simulink model "fix_FOC_sync"  (R2025b)
settings: Solver=FixedStepAuto  StartTime=0.0  StopTime=10.0  FixedStep=0.001  RelTol=1e-3
values from neighbouring files (symbols this model uses):
  Dm = 1e-3    (= 0.001)    [motor_param.m]
  Ki_id = wc_c*Rs    (= 380)    [motor_param.m]
  Ki_iq = wc_c*Rs    (= 380)    [motor_param.m]
  Ki_s = 0.041    [motor_param.m]
  Kp_id = wc_c*Ld    (= 10)    [motor_param.m]
  Kp_iq = wc_c*Lq    (= 20)    [motor_param.m]
  Kp_s = 0.0014    [motor_param.m]
  Ld = 0.01    [motor_param.m]
  Lq = 0.02    [motor_param.m]
  p = 2    [motor_param.m]
  Phi = 0.1    [motor_param.m]
libraries: fl_lib x50, nesl_utility x50, slpidlib x15, ee_lib x15, eeTransforms x10
(part 3 of 4)

== system fix_FOC_sync/Subsystem5/Plant/MechSensor ==
  Ideal Rotational Motion Sensor : fl_lib/Mechanical/Mechanical Sensors/Ideal Rotational Motion Sensor  reference=foundation.enum.MeasurementReference.difference  acceleration_port=false  velocity_port=true  position_port=true  wrap_angle=simscape.enum.onoff.off  offset=0 rad
  Ideal Torque Sensor : fl_lib/Mechanical/Mechanical Sensors/Ideal Torque Sensor
  PS-Simulink Converter : nesl_utility/PS-Simulink Converter  PhysicalDomain=network_engine_domain  SubClassName=ps_output  LeftPortType=input  RightPortType=output  PseudoPeriodic=off  Frequencies=[]  VectorFormat=1-D array  Unit=1  AffineConversion=off
  PS-Simulink Converter1 : nesl_utility/PS-Simulink Converter  PhysicalDomain=network_engine_domain  SubClassName=ps_output  LeftPortType=input  RightPortType=output  PseudoPeriodic=off  Frequencies=[]  VectorFormat=1-D array  Unit=1  AffineConversion=off
  PS-Simulink Converter2 : nesl_utility/PS-Simulink Converter  PhysicalDomain=network_engine_domain  SubClassName=ps_output  LeftPortType=input  RightPortType=output  PseudoPeriodic=off  Frequencies=[]  VectorFormat=1-D array  Unit=1  AffineConversion=off
  R1 : PMIOPort  Side=Left
  C1 : PMIOPort  Port=2  Side=Left
  R2 : PMIOPort  Port=3  Side=Right
  C2 : PMIOPort  Port=4  Side=Right
  wm : Outport  VectorParamsAs1DForOutWhenUnconnected=off
  thm : Outport  Port=2  VectorParamsAs1DForOutWhenUnconnected=off
  Tm : Outport  Port=3  VectorParamsAs1DForOutWhenUnconnected=off
  wires:
  PS-Simulink Converter/1 -> thm/1
  PS-Simulink Converter1/1 -> Tm/1
  PS-Simulink Converter2/1 -> wm/1
  connections:
  Ideal Rotational Motion Sensor/RConn3 -- PS-Simulink Converter/LConn1
  Ideal Rotational Motion Sensor/RConn1 -- C2/RConn1 -- C1/RConn1
  Ideal Torque Sensor/LConn1 -- R1/RConn1
  Ideal Torque Sensor/RConn1 -- R2/RConn1 -- Ideal Rotational Motion Sensor/LConn1
  PS-Simulink Converter1/LConn1 -- Ideal Torque Sensor/RConn2
  Ideal Rotational Motion Sensor/RConn2 -- PS-Simulink Converter2/LConn1

== system fix_FOC_sync/Subsystem1/Controller/DriverPeripherals/Break Algebraic Loop ==
  In1 : Inport
  Demux : Demux  Outputs=3
  Mux : Mux  Inputs=3
  Transfer Fcn : TransferFcn  Denominator=[1e-6 1]
  Transfer Fcn1 : TransferFcn  Denominator=[1e-6 1]
  Transfer Fcn2 : TransferFcn  Denominator=[1e-6 1]
  Out1 : Outport
  wires:
  In1/1 -> Demux/1
  Demux/1 -> Transfer Fcn/1
  Transfer Fcn/1 -> Mux/1
  Demux/2 -> Transfer Fcn1/1
  Transfer Fcn1/1 -> Mux/2
  Demux/3 -> Transfer Fcn2/1
  Transfer Fcn2/1 -> Mux/3
  Mux/1 -> Out1/1

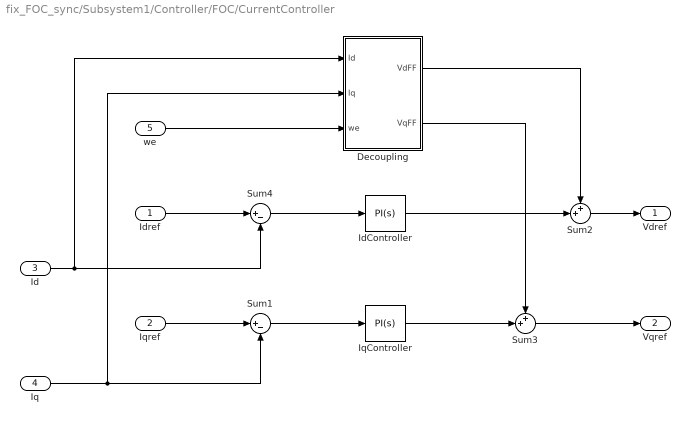
== system fix_FOC_sync/Subsystem1/Controller/FOC/CurrentController ==
  Idref : Inport
  Iqref : Inport  Port=2
  Id : Inport  Port=3
  Iq : Inport  Port=4
  we : Inport  Port=5
  Decoupling : Subsystem
  IdController : slpidlib/PID Controller  Controller=PI  Form=Parallel  TimeDomain=Continuous-time  UseExternalTs=off  SampleTime=-1  IntegratorMethod=Forward Euler  FilterMethod=Forward Euler  ControllerParametersSource=internal  P=Kp_id  I=Ki_id  UseKiTs=off  D=0  UseExternalDerivativeSource=off  N=100  UseFilter=on  TunerSelectOption=Transfer Function Based (PID Tuner App)  InitialConditionSource=internal  InitialConditionForIntegrator=0  InitialConditionForFilter=0  DifferentiatorICPrevScaledInput=0  ExternalReset=none  TrackingMode=off  Kt=1  LimitOutput=off  SatLimitsSource=internal  UpperSaturationLimit=inf  LowerSaturationLimit=-inf  LinearizeAsGain=on  AntiWindupMode=none  Kb=1  LimitIntegrator=off  UpperIntegratorSaturationLimit=inf  LowerIntegratorSaturationLimit=-inf  POutMin=[]  POutMax=[]  IOutMin=[]  IOutMax=[]  DOutMin=[]  DOutMax=[]  NOutMin=[]  NOutMax=[]  SumOutMin=[]  SumOutMax=[]  SaturationOutMin=[]  SaturationOutMax=[]  PParamMin=[]  PParamMax=[]  IParamMin=[]  IParamMax=[]  DParamMin=[]  DParamMax=[]  NParamMin=[]  NParamMax=[]  KbParamMin=[]  KbParamMax=[]  KtParamMin=[]  KtParamMax=[]  KbOutMin=[]  KbOutMax=[]  KtOutMin=[]  KtOutMax=[]  IntegratorOutMin=[]  IntegratorOutMax=[]  FilterOutMin=[]  FilterOutMax=[]  SumI1OutMin=[]  SumI1OutMax=[]  SumI2OutMin=[]  SumI2OutMax=[]  SumI3OutMin=[]  SumI3OutMax=[]  SumI4OutMin=[]  SumI4OutMax=[]  SumDOutMin=[]  SumDOutMax=[]  DifferentiatorOutMin=[]  DifferentiatorOutMax=[]  FilterDiffOutCoefMin=[]  FilterDiffOutCoefMax=[]  ReciprocalOutMin=[]  ReciprocalOutMax=[]  SumDenOutMin=[]  SumDenOutMax=[]  SumNumOutMin=[]  SumNumOutMax=[]  DivideOutMin=[]  DivideOutMax=[]  UdiffTsProdOutMin=[]  UdiffTsProdOutMax=[]  NTsProdOutMin=[]  NTsProdOutMax=[]  UintegralTsProdOutMin=[]  UintegralTsProdOutMax=[]  UngainTsProdOutMin=[]  UngainTsProdOutMax=[]  ClampingZeroOutDataTypeStr=Inherit: Inherit via back propagation  ClampingZeroOutMin=[]  ClampingZeroOutMax=[]  FilterDenConstantOutDataTypeStr=Inherit: Inherit via back propagation  FilterDenConstantOutMin=[]  FilterDenConstantOutMax=[]  PCopyOutDataTypeStr=Inherit: Inherit via back propagation  PCopyOutMin=[]  PCopyOutMax=[]  NCopyOutDataTypeStr=Inherit: Inherit via back propagation  NCopyOutMin=[]  NCopyOutMax=[]  IntegratorContinuousStateAttributes=''  IntegratorStateMustResolveToSignalObject=off  IntegratorRTWStateStorageClass=Auto  FilterContinuousStateAttributes=''  FilterStateMustResolveToSignalObject=off  FilterRTWStateStorageClass=Auto  ParallelPVariant=InternalParameters  IdealPVariant=Disabled  IVariant=InternalParameters  DVariant=Disabled  IntegratorVariant=Continuous  SatVariant=Disabled  AWVariant=Passthrough  PCopyVariant=Disabled  TRVariant=Disabled  FdbkBlocksVariant=Forward  IdealPFdbkVariant=Disabled  SatFdbkVariant=Disabled  DerivativeFilterVariant=Disabled  NVariant=Disabled  NCopyVariant=Disabled_SignalSpec  FilterICVariant=Disabled  IntegratorICVariant=InternalICs  ExternalResetVariant=Disabled  TRSumVariant=Passthrough  SumFdbkVariant=Disabled  SumVariant=Sum_PI  TsampFilterVariant=InternalTs  TsampNgainVariant=Passthrough  TsampIntegralVariant=Disabled_SignalSpec  ExternalSaturationOutDataTypeStr=Inherit: Same as second input  DerivativeSourceVariant=Disabled  PreIntVariant=InternalPreInt
  IqController : slpidlib/PID Controller  Controller=PI  Form=Parallel  TimeDomain=Continuous-time  UseExternalTs=off  SampleTime=-1  IntegratorMethod=Forward Euler  FilterMethod=Forward Euler  ControllerParametersSource=internal  P=Kp_iq  I=Ki_iq  UseKiTs=off  D=0  UseExternalDerivativeSource=off  N=100  UseFilter=on  TunerSelectOption=Transfer Function Based (PID Tuner App)  InitialConditionSource=internal  InitialConditionForIntegrator=0  InitialConditionForFilter=0  DifferentiatorICPrevScaledInput=0  ExternalReset=none  TrackingMode=off  Kt=1  LimitOutput=off  SatLimitsSource=internal  UpperSaturationLimit=inf  LowerSaturationLimit=-inf  LinearizeAsGain=on  AntiWindupMode=none  Kb=1  LimitIntegrator=off  UpperIntegratorSaturationLimit=inf  LowerIntegratorSaturationLimit=-inf  POutMin=[]  POutMax=[]  IOutMin=[]  IOutMax=[]  DOutMin=[]  DOutMax=[]  NOutMin=[]  NOutMax=[]  SumOutMin=[]  SumOutMax=[]  SaturationOutMin=[]  SaturationOutMax=[]  PParamMin=[]  PParamMax=[]  IParamMin=[]  IParamMax=[]  DParamMin=[]  DParamMax=[]  NParamMin=[]  NParamMax=[]  KbParamMin=[]  KbParamMax=[]  KtParamMin=[]  KtParamMax=[]  KbOutMin=[]  KbOutMax=[]  KtOutMin=[]  KtOutMax=[]  IntegratorOutMin=[]  IntegratorOutMax=[]  FilterOutMin=[]  FilterOutMax=[]  SumI1OutMin=[]  SumI1OutMax=[]  SumI2OutMin=[]  SumI2OutMax=[]  SumI3OutMin=[]  SumI3OutMax=[]  SumI4OutMin=[]  SumI4OutMax=[]  SumDOutMin=[]  SumDOutMax=[]  DifferentiatorOutMin=[]  DifferentiatorOutMax=[]  FilterDiffOutCoefMin=[]  FilterDiffOutCoefMax=[]  ReciprocalOutMin=[]  ReciprocalOutMax=[]  SumDenOutMin=[]  SumDenOutMax=[]  SumNumOutMin=[]  SumNumOutMax=[]  DivideOutMin=[]  DivideOutMax=[]  UdiffTsProdOutMin=[]  UdiffTsProdOutMax=[]  NTsProdOutMin=[]  NTsProdOutMax=[]  UintegralTsProdOutMin=[]  UintegralTsProdOutMax=[]  UngainTsProdOutMin=[]  UngainTsProdOutMax=[]  ClampingZeroOutDataTypeStr=Inherit: Inherit via back propagation  ClampingZeroOutMin=[]  ClampingZeroOutMax=[]  FilterDenConstantOutDataTypeStr=Inherit: Inherit via back propagation  FilterDenConstantOutMin=[]  FilterDenConstantOutMax=[]  PCopyOutDataTypeStr=Inherit: Inherit via back propagation  PCopyOutMin=[]  PCopyOutMax=[]  NCopyOutDataTypeStr=Inherit: Inherit via back propagation  NCopyOutMin=[]  NCopyOutMax=[]  IntegratorContinuousStateAttributes=''  IntegratorStateMustResolveToSignalObject=off  IntegratorRTWStateStorageClass=Auto  FilterContinuousStateAttributes=''  FilterStateMustResolveToSignalObject=off  FilterRTWStateStorageClass=Auto  ParallelPVariant=InternalParameters  IdealPVariant=Disabled  IVariant=InternalParameters  DVariant=Disabled  IntegratorVariant=Continuous  SatVariant=Disabled  AWVariant=Passthrough  PCopyVariant=Disabled  TRVariant=Disabled  FdbkBlocksVariant=Forward  IdealPFdbkVariant=Disabled  SatFdbkVariant=Disabled  DerivativeFilterVariant=Disabled  NVariant=Disabled  NCopyVariant=Disabled_SignalSpec  FilterICVariant=Disabled  IntegratorICVariant=InternalICs  ExternalResetVariant=Disabled  TRSumVariant=Passthrough  SumFdbkVariant=Disabled  SumVariant=Sum_PI  TsampFilterVariant=InternalTs  TsampNgainVariant=Passthrough  TsampIntegralVariant=Disabled_SignalSpec  ExternalSaturationOutDataTypeStr=Inherit: Same as second input  DerivativeSourceVariant=Disabled  PreIntVariant=InternalPreInt
  Sum1 : Sum  Inputs=|+-
  Sum2 : Sum  Inputs=++|
  Sum3 : Sum  Inputs=++|
  Sum4 : Sum  Inputs=|+-
  Vdref : Outport  VectorParamsAs1DForOutWhenUnconnected=off
  Vqref : Outport  Port=2  VectorParamsAs1DForOutWhenUnconnected=off
  wires:
  we/1 -> Decoupling/3(we)
  Idref/1 -> Sum4/1
  Sum2/1 -> Vdref/1
  Sum3/1 -> Vqref/1
  Iqref/1 -> Sum1/1
  Iq/1 -> Decoupling/2(Iq), Sum1/2
  Id/1 -> Decoupling/1(Id), Sum4/2
  Sum4/1 -> IdController/1
  Sum1/1 -> IqController/1
  Decoupling/2(VqFF) -> Sum3/1
  Decoupling/1(VdFF) -> Sum2/1
  IdController/1 -> Sum2/2
  IqController/1 -> Sum3/2

== system fix_FOC_sync/Subsystem1/Controller/FOC/VelocityController ==
  wmref : Inport
  wm : Inport  Port=2
  Gain : Gain  Gain=1/(3/2*p*Phi)
  PIDController : slpidlib/PID Controller  Controller=PI  Form=Parallel  TimeDomain=Continuous-time  UseExternalTs=off  SampleTime=-1  IntegratorMethod=Forward Euler  FilterMethod=Forward Euler  ControllerParametersSource=internal  P=Kp_s  I=Ki_s  UseKiTs=off  D=0  UseExternalDerivativeSource=off  N=100  UseFilter=on  TunerSelectOption=Transfer Function Based (PID Tuner App)  InitialConditionSource=internal  InitialConditionForIntegrator=0  InitialConditionForFilter=0  DifferentiatorICPrevScaledInput=0  ExternalReset=none  TrackingMode=off  Kt=1  LimitOutput=off  SatLimitsSource=internal  UpperSaturationLimit=inf  LowerSaturationLimit=-inf  LinearizeAsGain=on  AntiWindupMode=none  Kb=1  LimitIntegrator=off  UpperIntegratorSaturationLimit=inf  LowerIntegratorSaturationLimit=-inf  POutMin=[]  POutMax=[]  IOutMin=[]  IOutMax=[]  DOutMin=[]  DOutMax=[]  NOutMin=[]  NOutMax=[]  SumOutMin=[]  SumOutMax=[]  SaturationOutMin=[]  SaturationOutMax=[]  PParamMin=[]  PParamMax=[]  IParamMin=[]  IParamMax=[]  DParamMin=[]  DParamMax=[]  NParamMin=[]  NParamMax=[]  KbParamMin=[]  KbParamMax=[]  KtParamMin=[]  KtParamMax=[]  KbOutMin=[]  KbOutMax=[]  KtOutMin=[]  KtOutMax=[]  IntegratorOutMin=[]  IntegratorOutMax=[]  FilterOutMin=[]  FilterOutMax=[]  SumI1OutMin=[]  SumI1OutMax=[]  SumI2OutMin=[]  SumI2OutMax=[]  SumI3OutMin=[]  SumI3OutMax=[]  SumI4OutMin=[]  SumI4OutMax=[]  SumDOutMin=[]  SumDOutMax=[]  DifferentiatorOutMin=[]  DifferentiatorOutMax=[]  FilterDiffOutCoefMin=[]  FilterDiffOutCoefMax=[]  ReciprocalOutMin=[]  ReciprocalOutMax=[]  SumDenOutMin=[]  SumDenOutMax=[]  SumNumOutMin=[]  SumNumOutMax=[]  DivideOutMin=[]  DivideOutMax=[]  UdiffTsProdOutMin=[]  UdiffTsProdOutMax=[]  NTsProdOutMin=[]  NTsProdOutMax=[]  UintegralTsProdOutMin=[]  UintegralTsProdOutMax=[]  UngainTsProdOutMin=[]  UngainTsProdOutMax=[]  ClampingZeroOutDataTypeStr=Inherit: Inherit via back propagation  ClampingZeroOutMin=[]  ClampingZeroOutMax=[]  FilterDenConstantOutDataTypeStr=Inherit: Inherit via back propagation  FilterDenConstantOutMin=[]  FilterDenConstantOutMax=[]  PCopyOutDataTypeStr=Inherit: Inherit via back propagation  PCopyOutMin=[]  PCopyOutMax=[]  NCopyOutDataTypeStr=Inherit: Inherit via back propagation  NCopyOutMin=[]  NCopyOutMax=[]  IntegratorContinuousStateAttributes=''  IntegratorStateMustResolveToSignalObject=off  IntegratorRTWStateStorageClass=Auto  FilterContinuousStateAttributes=''  FilterStateMustResolveToSignalObject=off  FilterRTWStateStorageClass=Auto  ParallelPVariant=InternalParameters  IdealPVariant=Disabled  IVariant=InternalParameters  DVariant=Disabled  IntegratorVariant=Continuous  SatVariant=Disabled  AWVariant=Passthrough  PCopyVariant=Disabled  TRVariant=Disabled  FdbkBlocksVariant=Forward  IdealPFdbkVariant=Disabled  SatFdbkVariant=Disabled  DerivativeFilterVariant=Disabled  NVariant=Disabled  NCopyVariant=Disabled_SignalSpec  FilterICVariant=Disabled  IntegratorICVariant=InternalICs  ExternalResetVariant=Disabled  TRSumVariant=Passthrough  SumFdbkVariant=Disabled  SumVariant=Sum_PI  TsampFilterVariant=InternalTs  TsampNgainVariant=Passthrough  TsampIntegralVariant=Disabled_SignalSpec  ExternalSaturationOutDataTypeStr=Inherit: Same as second input  DerivativeSourceVariant=Disabled  PreIntVariant=InternalPreInt
  Sum : Sum  Inputs=|+-
  Iqref : Outport  VectorParamsAs1DForOutWhenUnconnected=off
  wires:
  Gain/1 -> Iqref/1
  wmref/1 -> Sum/1
  wm/1 -> Sum/2
  Sum/1 -> PIDController/1
  PIDController/1 -> Gain/1

== system fix_FOC_sync/Subsystem1/Controller/FOC/abc2dq ==
  Iabc : Inport
  thetae : Inport  Port=2
  Demux1 : Demux  Outputs=3
  Park Transform : eeTransforms/Park Transform  AxisAlignment=D-axis  PowerInvariant=off
  Terminator : Terminator
  Id : Outport  VectorParamsAs1DForOutWhenUnconnected=off
  Iq : Outport  Port=2  VectorParamsAs1DForOutWhenUnconnected=off
  wires:
  Iabc/1 -> Park Transform/1
  thetae/1 -> Park Transform/2
  Demux1/3 -> Terminator/1
  Park Transform/1 -> Demux1/1
  Demux1/1 -> Id/1
  Demux1/2 -> Iq/1

== system fix_FOC_sync/Subsystem1/Controller/FOC/dq2abc ==
  Vd : Inport
  Vq : Inport  Port=2
  thetae : Inport  Port=3
  Constant : Constant  Value=0
  Inverse Park Transform : eeTransforms/Inverse Park Transform  AxisAlignment=D-axis  PowerInvariant=off
  Mux : Mux  Inputs=3
  Vabc : Outport  VectorParamsAs1DForOutWhenUnconnected=off
  wires:
  thetae/1 -> Inverse Park Transform/2
  Constant/1 -> Mux/3
  Mux/1 -> Inverse Park Transform/1
  Vd/1 -> Mux/1
  Inverse Park Transform/1 -> Vabc/1
  Vq/1 -> Mux/2

== system fix_FOC_sync/Subsystem1/Controller/FOC/thm2the ==
  thm : Inport
  Constant : Constant  Value=2*pi
  Mod : Math  Operator=mod  SignedPower=on
  PolePairs : Gain  Gain=p
  the : Outport  VectorParamsAs1DForOutWhenUnconnected=off
  wires:
  Constant/1 -> Mod/2
  PolePairs/1 -> Mod/1
  Mod/1 -> the/1
  thm/1 -> PolePairs/1

== system fix_FOC_sync/Subsystem1/Controller/FOC/wm2we ==
  wm : Inport
  PolePairs : Gain  Gain=p
  we : Outport  VectorParamsAs1DForOutWhenUnconnected=off
  wires:
  wm/1 -> PolePairs/1
  PolePairs/1 -> we/1

== system fix_FOC_sync/Subsystem2/Controller/DriverPeripherals/Break Algebraic Loop ==
  In1 : Inport
  Demux : Demux  Outputs=3
  Mux : Mux  Inputs=3
  Transfer Fcn : TransferFcn  Denominator=[1e-6 1]
  Transfer Fcn1 : TransferFcn  Denominator=[1e-6 1]
  Transfer Fcn2 : TransferFcn  Denominator=[1e-6 1]
  Out1 : Outport
  wires:
  In1/1 -> Demux/1
  Demux/1 -> Transfer Fcn/1
  Transfer Fcn/1 -> Mux/1
  Demux/2 -> Transfer Fcn1/1
  Transfer Fcn1/1 -> Mux/2
  Demux/3 -> Transfer Fcn2/1
  Transfer Fcn2/1 -> Mux/3
  Mux/1 -> Out1/1

== system fix_FOC_sync/Subsystem2/Controller/FOC/CurrentController ==
  Idref : Inport
  Iqref : Inport  Port=2
  Id : Inport  Port=3
  Iq : Inport  Port=4
  we : Inport  Port=5
  Decoupling : Subsystem
  IdController : slpidlib/PID Controller  Controller=PI  Form=Parallel  TimeDomain=Continuous-time  UseExternalTs=off  SampleTime=-1  IntegratorMethod=Forward Euler  FilterMethod=Forward Euler  ControllerParametersSource=internal  P=Kp_id  I=Ki_id  UseKiTs=off  D=0  UseExternalDerivativeSource=off  N=100  UseFilter=on  TunerSelectOption=Transfer Function Based (PID Tuner App)  InitialConditionSource=internal  InitialConditionForIntegrator=0  InitialConditionForFilter=0  DifferentiatorICPrevScaledInput=0  ExternalReset=none  TrackingMode=off  Kt=1  LimitOutput=off  SatLimitsSource=internal  UpperSaturationLimit=inf  LowerSaturationLimit=-inf  LinearizeAsGain=on  AntiWindupMode=none  Kb=1  LimitIntegrator=off  UpperIntegratorSaturationLimit=inf  LowerIntegratorSaturationLimit=-inf  POutMin=[]  POutMax=[]  IOutMin=[]  IOutMax=[]  DOutMin=[]  DOutMax=[]  NOutMin=[]  NOutMax=[]  SumOutMin=[]  SumOutMax=[]  SaturationOutMin=[]  SaturationOutMax=[]  PParamMin=[]  PParamMax=[]  IParamMin=[]  IParamMax=[]  DParamMin=[]  DParamMax=[]  NParamMin=[]  NParamMax=[]  KbParamMin=[]  KbParamMax=[]  KtParamMin=[]  KtParamMax=[]  KbOutMin=[]  KbOutMax=[]  KtOutMin=[]  KtOutMax=[]  IntegratorOutMin=[]  IntegratorOutMax=[]  FilterOutMin=[]  FilterOutMax=[]  SumI1OutMin=[]  SumI1OutMax=[]  SumI2OutMin=[]  SumI2OutMax=[]  SumI3OutMin=[]  SumI3OutMax=[]  SumI4OutMin=[]  SumI4OutMax=[]  SumDOutMin=[]  SumDOutMax=[]  DifferentiatorOutMin=[]  DifferentiatorOutMax=[]  FilterDiffOutCoefMin=[]  FilterDiffOutCoefMax=[]  ReciprocalOutMin=[]  ReciprocalOutMax=[]  SumDenOutMin=[]  SumDenOutMax=[]  SumNumOutMin=[]  SumNumOutMax=[]  DivideOutMin=[]  DivideOutMax=[]  UdiffTsProdOutMin=[]  UdiffTsProdOutMax=[]  NTsProdOutMin=[]  NTsProdOutMax=[]  UintegralTsProdOutMin=[]  UintegralTsProdOutMax=[]  UngainTsProdOutMin=[]  UngainTsProdOutMax=[]  ClampingZeroOutDataTypeStr=Inherit: Inherit via back propagation  ClampingZeroOutMin=[]  ClampingZeroOutMax=[]  FilterDenConstantOutDataTypeStr=Inherit: Inherit via back propagation  FilterDenConstantOutMin=[]  FilterDenConstantOutMax=[]  PCopyOutDataTypeStr=Inherit: Inherit via back propagation  PCopyOutMin=[]  PCopyOutMax=[]  NCopyOutDataTypeStr=Inherit: Inherit via back propagation  NCopyOutMin=[]  NCopyOutMax=[]  IntegratorContinuousStateAttributes=''  IntegratorStateMustResolveToSignalObject=off  IntegratorRTWStateStorageClass=Auto  FilterContinuousStateAttributes=''  FilterStateMustResolveToSignalObject=off  FilterRTWStateStorageClass=Auto  ParallelPVariant=InternalParameters  IdealPVariant=Disabled  IVariant=InternalParameters  DVariant=Disabled  IntegratorVariant=Continuous  SatVariant=Disabled  AWVariant=Passthrough  PCopyVariant=Disabled  TRVariant=Disabled  FdbkBlocksVariant=Forward  IdealPFdbkVariant=Disabled  SatFdbkVariant=Disabled  DerivativeFilterVariant=Disabled  NVariant=Disabled  NCopyVariant=Disabled_SignalSpec  FilterICVariant=Disabled  IntegratorICVariant=InternalICs  ExternalResetVariant=Disabled  TRSumVariant=Passthrough  SumFdbkVariant=Disabled  SumVariant=Sum_PI  TsampFilterVariant=InternalTs  TsampNgainVariant=Passthrough  TsampIntegralVariant=Disabled_SignalSpec  ExternalSaturationOutDataTypeStr=Inherit: Same as second input  DerivativeSourceVariant=Disabled  PreIntVariant=InternalPreInt
  IqController : slpidlib/PID Controller  Controller=PI  Form=Parallel  TimeDomain=Continuous-time  UseExternalTs=off  SampleTime=-1  IntegratorMethod=Forward Euler  FilterMethod=Forward Euler  ControllerParametersSource=internal  P=Kp_iq  I=Ki_iq  UseKiTs=off  D=0  UseExternalDerivativeSource=off  N=100  UseFilter=on  TunerSelectOption=Transfer Function Based (PID Tuner App)  InitialConditionSource=internal  InitialConditionForIntegrator=0  InitialConditionForFilter=0  DifferentiatorICPrevScaledInput=0  ExternalReset=none  TrackingMode=off  Kt=1  LimitOutput=off  SatLimitsSource=internal  UpperSaturationLimit=inf  LowerSaturationLimit=-inf  LinearizeAsGain=on  AntiWindupMode=none  Kb=1  LimitIntegrator=off  UpperIntegratorSaturationLimit=inf  LowerIntegratorSaturationLimit=-inf  POutMin=[]  POutMax=[]  IOutMin=[]  IOutMax=[]  DOutMin=[]  DOutMax=[]  NOutMin=[]  NOutMax=[]  SumOutMin=[]  SumOutMax=[]  SaturationOutMin=[]  SaturationOutMax=[]  PParamMin=[]  PParamMax=[]  IParamMin=[]  IParamMax=[]  DParamMin=[]  DParamMax=[]  NParamMin=[]  NParamMax=[]  KbParamMin=[]  KbParamMax=[]  KtParamMin=[]  KtParamMax=[]  KbOutMin=[]  KbOutMax=[]  KtOutMin=[]  KtOutMax=[]  IntegratorOutMin=[]  IntegratorOutMax=[]  FilterOutMin=[]  FilterOutMax=[]  SumI1OutMin=[]  SumI1OutMax=[]  SumI2OutMin=[]  SumI2OutMax=[]  SumI3OutMin=[]  SumI3OutMax=[]  SumI4OutMin=[]  SumI4OutMax=[]  SumDOutMin=[]  SumDOutMax=[]  DifferentiatorOutMin=[]  DifferentiatorOutMax=[]  FilterDiffOutCoefMin=[]  FilterDiffOutCoefMax=[]  ReciprocalOutMin=[]  ReciprocalOutMax=[]  SumDenOutMin=[]  SumDenOutMax=[]  SumNumOutMin=[]  SumNumOutMax=[]  DivideOutMin=[]  DivideOutMax=[]  UdiffTsProdOutMin=[]  UdiffTsProdOutMax=[]  NTsProdOutMin=[]  NTsProdOutMax=[]  UintegralTsProdOutMin=[]  UintegralTsProdOutMax=[]  UngainTsProdOutMin=[]  UngainTsProdOutMax=[]  ClampingZeroOutDataTypeStr=Inherit: Inherit via back propagation  ClampingZeroOutMin=[]  ClampingZeroOutMax=[]  FilterDenConstantOutDataTypeStr=Inherit: Inherit via back propagation  FilterDenConstantOutMin=[]  FilterDenConstantOutMax=[]  PCopyOutDataTypeStr=Inherit: Inherit via back propagation  PCopyOutMin=[]  PCopyOutMax=[]  NCopyOutDataTypeStr=Inherit: Inherit via back propagation  NCopyOutMin=[]  NCopyOutMax=[]  IntegratorContinuousStateAttributes=''  IntegratorStateMustResolveToSignalObject=off  IntegratorRTWStateStorageClass=Auto  FilterContinuousStateAttributes=''  FilterStateMustResolveToSignalObject=off  FilterRTWStateStorageClass=Auto  ParallelPVariant=InternalParameters  IdealPVariant=Disabled  IVariant=InternalParameters  DVariant=Disabled  IntegratorVariant=Continuous  SatVariant=Disabled  AWVariant=Passthrough  PCopyVariant=Disabled  TRVariant=Disabled  FdbkBlocksVariant=Forward  IdealPFdbkVariant=Disabled  SatFdbkVariant=Disabled  DerivativeFilterVariant=Disabled  NVariant=Disabled  NCopyVariant=Disabled_SignalSpec  FilterICVariant=Disabled  IntegratorICVariant=InternalICs  ExternalResetVariant=Disabled  TRSumVariant=Passthrough  SumFdbkVariant=Disabled  SumVariant=Sum_PI  TsampFilterVariant=InternalTs  TsampNgainVariant=Passthrough  TsampIntegralVariant=Disabled_SignalSpec  ExternalSaturationOutDataTypeStr=Inherit: Same as second input  DerivativeSourceVariant=Disabled  PreIntVariant=InternalPreInt
  Sum1 : Sum  Inputs=|+-
  Sum2 : Sum  Inputs=++|
  Sum3 : Sum  Inputs=++|
  Sum4 : Sum  Inputs=|+-
  Vdref : Outport  VectorParamsAs1DForOutWhenUnconnected=off
  Vqref : Outport  Port=2  VectorParamsAs1DForOutWhenUnconnected=off
  wires:
  we/1 -> Decoupling/3(we)
  Idref/1 -> Sum4/1
  Sum2/1 -> Vdref/1
  Sum3/1 -> Vqref/1
  Iqref/1 -> Sum1/1
  Iq/1 -> Decoupling/2(Iq), Sum1/2
  Id/1 -> Decoupling/1(Id), Sum4/2
  Sum4/1 -> IdController/1
  Sum1/1 -> IqController/1
  Decoupling/2(VqFF) -> Sum3/1
  Decoupling/1(VdFF) -> Sum2/1
  IdController/1 -> Sum2/2
  IqController/1 -> Sum3/2

== system fix_FOC_sync/Subsystem2/Controller/FOC/VelocityController ==
  wmref : Inport
  wm : Inport  Port=2
  Gain : Gain  Gain=1/(3/2*p*Phi)
  PIDController : slpidlib/PID Controller  Controller=PI  Form=Parallel  TimeDomain=Continuous-time  UseExternalTs=off  SampleTime=-1  IntegratorMethod=Forward Euler  FilterMethod=Forward Euler  ControllerParametersSource=internal  P=Kp_s  I=Ki_s  UseKiTs=off  D=0  UseExternalDerivativeSource=off  N=100  UseFilter=on  TunerSelectOption=Transfer Function Based (PID Tuner App)  InitialConditionSource=internal  InitialConditionForIntegrator=0  InitialConditionForFilter=0  DifferentiatorICPrevScaledInput=0  ExternalReset=none  TrackingMode=off  Kt=1  LimitOutput=off  SatLimitsSource=internal  UpperSaturationLimit=inf  LowerSaturationLimit=-inf  LinearizeAsGain=on  AntiWindupMode=none  Kb=1  LimitIntegrator=off  UpperIntegratorSaturationLimit=inf  LowerIntegratorSaturationLimit=-inf  POutMin=[]  POutMax=[]  IOutMin=[]  IOutMax=[]  DOutMin=[]  DOutMax=[]  NOutMin=[]  NOutMax=[]  SumOutMin=[]  SumOutMax=[]  SaturationOutMin=[]  SaturationOutMax=[]  PParamMin=[]  PParamMax=[]  IParamMin=[]  IParamMax=[]  DParamMin=[]  DParamMax=[]  NParamMin=[]  NParamMax=[]  KbParamMin=[]  KbParamMax=[]  KtParamMin=[]  KtParamMax=[]  KbOutMin=[]  KbOutMax=[]  KtOutMin=[]  KtOutMax=[]  IntegratorOutMin=[]  IntegratorOutMax=[]  FilterOutMin=[]  FilterOutMax=[]  SumI1OutMin=[]  SumI1OutMax=[]  SumI2OutMin=[]  SumI2OutMax=[]  SumI3OutMin=[]  SumI3OutMax=[]  SumI4OutMin=[]  SumI4OutMax=[]  SumDOutMin=[]  SumDOutMax=[]  DifferentiatorOutMin=[]  DifferentiatorOutMax=[]  FilterDiffOutCoefMin=[]  FilterDiffOutCoefMax=[]  ReciprocalOutMin=[]  ReciprocalOutMax=[]  SumDenOutMin=[]  SumDenOutMax=[]  SumNumOutMin=[]  SumNumOutMax=[]  DivideOutMin=[]  DivideOutMax=[]  UdiffTsProdOutMin=[]  UdiffTsProdOutMax=[]  NTsProdOutMin=[]  NTsProdOutMax=[]  UintegralTsProdOutMin=[]  UintegralTsProdOutMax=[]  UngainTsProdOutMin=[]  UngainTsProdOutMax=[]  ClampingZeroOutDataTypeStr=Inherit: Inherit via back propagation  ClampingZeroOutMin=[]  ClampingZeroOutMax=[]  FilterDenConstantOutDataTypeStr=Inherit: Inherit via back propagation  FilterDenConstantOutMin=[]  FilterDenConstantOutMax=[]  PCopyOutDataTypeStr=Inherit: Inherit via back propagation  PCopyOutMin=[]  PCopyOutMax=[]  NCopyOutDataTypeStr=Inherit: Inherit via back propagation  NCopyOutMin=[]  NCopyOutMax=[]  IntegratorContinuousStateAttributes=''  IntegratorStateMustResolveToSignalObject=off  IntegratorRTWStateStorageClass=Auto  FilterContinuousStateAttributes=''  FilterStateMustResolveToSignalObject=off  FilterRTWStateStorageClass=Auto  ParallelPVariant=InternalParameters  IdealPVariant=Disabled  IVariant=InternalParameters  DVariant=Disabled  IntegratorVariant=Continuous  SatVariant=Disabled  AWVariant=Passthrough  PCopyVariant=Disabled  TRVariant=Disabled  FdbkBlocksVariant=Forward  IdealPFdbkVariant=Disabled  SatFdbkVariant=Disabled  DerivativeFilterVariant=Disabled  NVariant=Disabled  NCopyVariant=Disabled_SignalSpec  FilterICVariant=Disabled  IntegratorICVariant=InternalICs  ExternalResetVariant=Disabled  TRSumVariant=Passthrough  SumFdbkVariant=Disabled  SumVariant=Sum_PI  TsampFilterVariant=InternalTs  TsampNgainVariant=Passthrough  TsampIntegralVariant=Disabled_SignalSpec  ExternalSaturationOutDataTypeStr=Inherit: Same as second input  DerivativeSourceVariant=Disabled  PreIntVariant=InternalPreInt
  Sum : Sum  Inputs=|+-
  Iqref : Outport  VectorParamsAs1DForOutWhenUnconnected=off
  wires:
  PIDController/1 -> Gain/1
  Gain/1 -> Iqref/1
  wmref/1 -> Sum/1
  Sum/1 -> PIDController/1
  wm/1 -> Sum/2

== system fix_FOC_sync/Subsystem2/Controller/FOC/abc2dq ==
  Iabc : Inport
  thetae : Inport  Port=2
  Demux1 : Demux  Outputs=3
  Park Transform : eeTransforms/Park Transform  AxisAlignment=D-axis  PowerInvariant=off
  Terminator : Terminator
  Id : Outport  VectorParamsAs1DForOutWhenUnconnected=off
  Iq : Outport  Port=2  VectorParamsAs1DForOutWhenUnconnected=off
  wires:
  Iabc/1 -> Park Transform/1
  thetae/1 -> Park Transform/2
  Demux1/3 -> Terminator/1
  Park Transform/1 -> Demux1/1
  Demux1/1 -> Id/1
  Demux1/2 -> Iq/1

== system fix_FOC_sync/Subsystem2/Controller/FOC/dq2abc ==
  Vd : Inport
  Vq : Inport  Port=2
  thetae : Inport  Port=3
  Constant : Constant  Value=0
  Inverse Park Transform : eeTransforms/Inverse Park Transform  AxisAlignment=D-axis  PowerInvariant=off
  Mux : Mux  Inputs=3
  Vabc : Outport  VectorParamsAs1DForOutWhenUnconnected=off
  wires:
  thetae/1 -> Inverse Park Transform/2
  Constant/1 -> Mux/3
  Mux/1 -> Inverse Park Transform/1
  Vd/1 -> Mux/1
  Inverse Park Transform/1 -> Vabc/1
  Vq/1 -> Mux/2

== system fix_FOC_sync/Subsystem2/Controller/FOC/thm2the ==
  thm : Inport
  Constant : Constant  Value=2*pi
  Mod : Math  Operator=mod  SignedPower=on
  PolePairs : Gain  Gain=p
  the : Outport  VectorParamsAs1DForOutWhenUnconnected=off
  wires:
  Constant/1 -> Mod/2
  PolePairs/1 -> Mod/1
  Mod/1 -> the/1
  thm/1 -> PolePairs/1

== system fix_FOC_sync/Subsystem2/Controller/FOC/wm2we ==
  wm : Inport
  PolePairs : Gain  Gain=p
  we : Outport  VectorParamsAs1DForOutWhenUnconnected=off
  wires:
  wm/1 -> PolePairs/1
  PolePairs/1 -> we/1

== system fix_FOC_sync/Subsystem3/Controller/DriverPeripherals/Break Algebraic Loop ==
  In1 : Inport
  Demux : Demux  Outputs=3
  Mux : Mux  Inputs=3
  Transfer Fcn : TransferFcn  Denominator=[1e-6 1]
  Transfer Fcn1 : TransferFcn  Denominator=[1e-6 1]
  Transfer Fcn2 : TransferFcn  Denominator=[1e-6 1]
  Out1 : Outport
  wires:
  In1/1 -> Demux/1
  Demux/1 -> Transfer Fcn/1
  Transfer Fcn/1 -> Mux/1
  Demux/2 -> Transfer Fcn1/1
  Transfer Fcn1/1 -> Mux/2
  Demux/3 -> Transfer Fcn2/1
  Transfer Fcn2/1 -> Mux/3
  Mux/1 -> Out1/1

== system fix_FOC_sync/Subsystem3/Controller/FOC/CurrentController ==
  Idref : Inport
  Iqref : Inport  Port=2
  Id : Inport  Port=3
  Iq : Inport  Port=4
  we : Inport  Port=5
  Decoupling : Subsystem
  IdController : slpidlib/PID Controller  Controller=PI  Form=Parallel  TimeDomain=Continuous-time  UseExternalTs=off  SampleTime=-1  IntegratorMethod=Forward Euler  FilterMethod=Forward Euler  ControllerParametersSource=internal  P=Kp_id  I=Ki_id  UseKiTs=off  D=0  UseExternalDerivativeSource=off  N=100  UseFilter=on  TunerSelectOption=Transfer Function Based (PID Tuner App)  InitialConditionSource=internal  InitialConditionForIntegrator=0  InitialConditionForFilter=0  DifferentiatorICPrevScaledInput=0  ExternalReset=none  TrackingMode=off  Kt=1  LimitOutput=off  SatLimitsSource=internal  UpperSaturationLimit=inf  LowerSaturationLimit=-inf  LinearizeAsGain=on  AntiWindupMode=none  Kb=1  LimitIntegrator=off  UpperIntegratorSaturationLimit=inf  LowerIntegratorSaturationLimit=-inf  POutMin=[]  POutMax=[]  IOutMin=[]  IOutMax=[]  DOutMin=[]  DOutMax=[]  NOutMin=[]  NOutMax=[]  SumOutMin=[]  SumOutMax=[]  SaturationOutMin=[]  SaturationOutMax=[]  PParamMin=[]  PParamMax=[]  IParamMin=[]  IParamMax=[]  DParamMin=[]  DParamMax=[]  NParamMin=[]  NParamMax=[]  KbParamMin=[]  KbParamMax=[]  KtParamMin=[]  KtParamMax=[]  KbOutMin=[]  KbOutMax=[]  KtOutMin=[]  KtOutMax=[]  IntegratorOutMin=[]  IntegratorOutMax=[]  FilterOutMin=[]  FilterOutMax=[]  SumI1OutMin=[]  SumI1OutMax=[]  SumI2OutMin=[]  SumI2OutMax=[]  SumI3OutMin=[]  SumI3OutMax=[]  SumI4OutMin=[]  SumI4OutMax=[]  SumDOutMin=[]  SumDOutMax=[]  DifferentiatorOutMin=[]  DifferentiatorOutMax=[]  FilterDiffOutCoefMin=[]  FilterDiffOutCoefMax=[]  ReciprocalOutMin=[]  ReciprocalOutMax=[]  SumDenOutMin=[]  SumDenOutMax=[]  SumNumOutMin=[]  SumNumOutMax=[]  DivideOutMin=[]  DivideOutMax=[]  UdiffTsProdOutMin=[]  UdiffTsProdOutMax=[]  NTsProdOutMin=[]  NTsProdOutMax=[]  UintegralTsProdOutMin=[]  UintegralTsProdOutMax=[]  UngainTsProdOutMin=[]  UngainTsProdOutMax=[]  ClampingZeroOutDataTypeStr=Inherit: Inherit via back propagation  ClampingZeroOutMin=[]  ClampingZeroOutMax=[]  FilterDenConstantOutDataTypeStr=Inherit: Inherit via back propagation  FilterDenConstantOutMin=[]  FilterDenConstantOutMax=[]  PCopyOutDataTypeStr=Inherit: Inherit via back propagation  PCopyOutMin=[]  PCopyOutMax=[]  NCopyOutDataTypeStr=Inherit: Inherit via back propagation  NCopyOutMin=[]  NCopyOutMax=[]  IntegratorContinuousStateAttributes=''  IntegratorStateMustResolveToSignalObject=off  IntegratorRTWStateStorageClass=Auto  FilterContinuousStateAttributes=''  FilterStateMustResolveToSignalObject=off  FilterRTWStateStorageClass=Auto  ParallelPVariant=InternalParameters  IdealPVariant=Disabled  IVariant=InternalParameters  DVariant=Disabled  IntegratorVariant=Continuous  SatVariant=Disabled  AWVariant=Passthrough  PCopyVariant=Disabled  TRVariant=Disabled  FdbkBlocksVariant=Forward  IdealPFdbkVariant=Disabled  SatFdbkVariant=Disabled  DerivativeFilterVariant=Disabled  NVariant=Disabled  NCopyVariant=Disabled_SignalSpec  FilterICVariant=Disabled  IntegratorICVariant=InternalICs  ExternalResetVariant=Disabled  TRSumVariant=Passthrough  SumFdbkVariant=Disabled  SumVariant=Sum_PI  TsampFilterVariant=InternalTs  TsampNgainVariant=Passthrough  TsampIntegralVariant=Disabled_SignalSpec  ExternalSaturationOutDataTypeStr=Inherit: Same as second input  DerivativeSourceVariant=Disabled  PreIntVariant=InternalPreInt
  IqController : slpidlib/PID Controller  Controller=PI  Form=Parallel  TimeDomain=Continuous-time  UseExternalTs=off  SampleTime=-1  IntegratorMethod=Forward Euler  FilterMethod=Forward Euler  ControllerParametersSource=internal  P=Kp_iq  I=Ki_iq  UseKiTs=off  D=0  UseExternalDerivativeSource=off  N=100  UseFilter=on  TunerSelectOption=Transfer Function Based (PID Tuner App)  InitialConditionSource=internal  InitialConditionForIntegrator=0  InitialConditionForFilter=0  DifferentiatorICPrevScaledInput=0  ExternalReset=none  TrackingMode=off  Kt=1  LimitOutput=off  SatLimitsSource=internal  UpperSaturationLimit=inf  LowerSaturationLimit=-inf  LinearizeAsGain=on  AntiWindupMode=none  Kb=1  LimitIntegrator=off  UpperIntegratorSaturationLimit=inf  LowerIntegratorSaturationLimit=-inf  POutMin=[]  POutMax=[]  IOutMin=[]  IOutMax=[]  DOutMin=[]  DOutMax=[]  NOutMin=[]  NOutMax=[]  SumOutMin=[]  SumOutMax=[]  SaturationOutMin=[]  SaturationOutMax=[]  PParamMin=[]  PParamMax=[]  IParamMin=[]  IParamMax=[]  DParamMin=[]  DParamMax=[]  NParamMin=[]  NParamMax=[]  KbParamMin=[]  KbParamMax=[]  KtParamMin=[]  KtParamMax=[]  KbOutMin=[]  KbOutMax=[]  KtOutMin=[]  KtOutMax=[]  IntegratorOutMin=[]  IntegratorOutMax=[]  FilterOutMin=[]  FilterOutMax=[]  SumI1OutMin=[]  SumI1OutMax=[]  SumI2OutMin=[]  SumI2OutMax=[]  SumI3OutMin=[]  SumI3OutMax=[]  SumI4OutMin=[]  SumI4OutMax=[]  SumDOutMin=[]  SumDOutMax=[]  DifferentiatorOutMin=[]  DifferentiatorOutMax=[]  FilterDiffOutCoefMin=[]  FilterDiffOutCoefMax=[]  ReciprocalOutMin=[]  ReciprocalOutMax=[]  SumDenOutMin=[]  SumDenOutMax=[]  SumNumOutMin=[]  SumNumOutMax=[]  DivideOutMin=[]  DivideOutMax=[]  UdiffTsProdOutMin=[]  UdiffTsProdOutMax=[]  NTsProdOutMin=[]  NTsProdOutMax=[]  UintegralTsProdOutMin=[]  UintegralTsProdOutMax=[]  UngainTsProdOutMin=[]  UngainTsProdOutMax=[]  ClampingZeroOutDataTypeStr=Inherit: Inherit via back propagation  ClampingZeroOutMin=[]  ClampingZeroOutMax=[]  FilterDenConstantOutDataTypeStr=Inherit: Inherit via back propagation  FilterDenConstantOutMin=[]  FilterDenConstantOutMax=[]  PCopyOutDataTypeStr=Inherit: Inherit via back propagation  PCopyOutMin=[]  PCopyOutMax=[]  NCopyOutDataTypeStr=Inherit: Inherit via back propagation  NCopyOutMin=[]  NCopyOutMax=[]  IntegratorContinuousStateAttributes=''  IntegratorStateMustResolveToSignalObject=off  IntegratorRTWStateStorageClass=Auto  FilterContinuousStateAttributes=''  FilterStateMustResolveToSignalObject=off  FilterRTWStateStorageClass=Auto  ParallelPVariant=InternalParameters  IdealPVariant=Disabled  IVariant=InternalParameters  DVariant=Disabled  IntegratorVariant=Continuous  SatVariant=Disabled  AWVariant=Passthrough  PCopyVariant=Disabled  TRVariant=Disabled  FdbkBlocksVariant=Forward  IdealPFdbkVariant=Disabled  SatFdbkVariant=Disabled  DerivativeFilterVariant=Disabled  NVariant=Disabled  NCopyVariant=Disabled_SignalSpec  FilterICVariant=Disabled  IntegratorICVariant=InternalICs  ExternalResetVariant=Disabled  TRSumVariant=Passthrough  SumFdbkVariant=Disabled  SumVariant=Sum_PI  TsampFilterVariant=InternalTs  TsampNgainVariant=Passthrough  TsampIntegralVariant=Disabled_SignalSpec  ExternalSaturationOutDataTypeStr=Inherit: Same as second input  DerivativeSourceVariant=Disabled  PreIntVariant=InternalPreInt
  Sum1 : Sum  Inputs=|+-
  Sum2 : Sum  Inputs=++|
  Sum3 : Sum  Inputs=++|
  Sum4 : Sum  Inputs=|+-
  Vdref : Outport  VectorParamsAs1DForOutWhenUnconnected=off
  Vqref : Outport  Port=2  VectorParamsAs1DForOutWhenUnconnected=off
  wires:
  we/1 -> Decoupling/3(we)
  Idref/1 -> Sum4/1
  Sum2/1 -> Vdref/1
  Sum3/1 -> Vqref/1
  Iqref/1 -> Sum1/1
  Iq/1 -> Decoupling/2(Iq), Sum1/2
  Id/1 -> Decoupling/1(Id), Sum4/2
  Sum4/1 -> IdController/1
  Sum1/1 -> IqController/1
  Decoupling/2(VqFF) -> Sum3/1
  Decoupling/1(VdFF) -> Sum2/1
  IdController/1 -> Sum2/2
  IqController/1 -> Sum3/2

== system fix_FOC_sync/Subsystem3/Controller/FOC/VelocityController ==
  wmref : Inport
  wm : Inport  Port=2
  Gain : Gain  Gain=1/(3/2*p*Phi)
  PIDController : slpidlib/PID Controller  Controller=PI  Form=Parallel  TimeDomain=Continuous-time  UseExternalTs=off  SampleTime=-1  IntegratorMethod=Forward Euler  FilterMethod=Forward Euler  ControllerParametersSource=internal  P=Kp_s  I=Ki_s  UseKiTs=off  D=0  UseExternalDerivativeSource=off  N=100  UseFilter=on  TunerSelectOption=Transfer Function Based (PID Tuner App)  InitialConditionSource=internal  InitialConditionForIntegrator=0  InitialConditionForFilter=0  DifferentiatorICPrevScaledInput=0  ExternalReset=none  TrackingMode=off  Kt=1  LimitOutput=off  SatLimitsSource=internal  UpperSaturationLimit=inf  LowerSaturationLimit=-inf  LinearizeAsGain=on  AntiWindupMode=none  Kb=1  LimitIntegrator=off  UpperIntegratorSaturationLimit=inf  LowerIntegratorSaturationLimit=-inf  POutMin=[]  POutMax=[]  IOutMin=[]  IOutMax=[]  DOutMin=[]  DOutMax=[]  NOutMin=[]  NOutMax=[]  SumOutMin=[]  SumOutMax=[]  SaturationOutMin=[]  SaturationOutMax=[]  PParamMin=[]  PParamMax=[]  IParamMin=[]  IParamMax=[]  DParamMin=[]  DParamMax=[]  NParamMin=[]  NParamMax=[]  KbParamMin=[]  KbParamMax=[]  KtParamMin=[]  KtParamMax=[]  KbOutMin=[]  KbOutMax=[]  KtOutMin=[]  KtOutMax=[]  IntegratorOutMin=[]  IntegratorOutMax=[]  FilterOutMin=[]  FilterOutMax=[]  SumI1OutMin=[]  SumI1OutMax=[]  SumI2OutMin=[]  SumI2OutMax=[]  SumI3OutMin=[]  SumI3OutMax=[]  SumI4OutMin=[]  SumI4OutMax=[]  SumDOutMin=[]  SumDOutMax=[]  DifferentiatorOutMin=[]  DifferentiatorOutMax=[]  FilterDiffOutCoefMin=[]  FilterDiffOutCoefMax=[]  ReciprocalOutMin=[]  ReciprocalOutMax=[]  SumDenOutMin=[]  SumDenOutMax=[]  SumNumOutMin=[]  SumNumOutMax=[]  DivideOutMin=[]  DivideOutMax=[]  UdiffTsProdOutMin=[]  UdiffTsProdOutMax=[]  NTsProdOutMin=[]  NTsProdOutMax=[]  UintegralTsProdOutMin=[]  UintegralTsProdOutMax=[]  UngainTsProdOutMin=[]  UngainTsProdOutMax=[]  ClampingZeroOutDataTypeStr=Inherit: Inherit via back propagation  ClampingZeroOutMin=[]  ClampingZeroOutMax=[]  FilterDenConstantOutDataTypeStr=Inherit: Inherit via back propagation  FilterDenConstantOutMin=[]  FilterDenConstantOutMax=[]  PCopyOutDataTypeStr=Inherit: Inherit via back propagation  PCopyOutMin=[]  PCopyOutMax=[]  NCopyOutDataTypeStr=Inherit: Inherit via back propagation  NCopyOutMin=[]  NCopyOutMax=[]  IntegratorContinuousStateAttributes=''  IntegratorStateMustResolveToSignalObject=off  IntegratorRTWStateStorageClass=Auto  FilterContinuousStateAttributes=''  FilterStateMustResolveToSignalObject=off  FilterRTWStateStorageClass=Auto  ParallelPVariant=InternalParameters  IdealPVariant=Disabled  IVariant=InternalParameters  DVariant=Disabled  IntegratorVariant=Continuous  SatVariant=Disabled  AWVariant=Passthrough  PCopyVariant=Disabled  TRVariant=Disabled  FdbkBlocksVariant=Forward  IdealPFdbkVariant=Disabled  SatFdbkVariant=Disabled  DerivativeFilterVariant=Disabled  NVariant=Disabled  NCopyVariant=Disabled_SignalSpec  FilterICVariant=Disabled  IntegratorICVariant=InternalICs  ExternalResetVariant=Disabled  TRSumVariant=Passthrough  SumFdbkVariant=Disabled  SumVariant=Sum_PI  TsampFilterVariant=InternalTs  TsampNgainVariant=Passthrough  TsampIntegralVariant=Disabled_SignalSpec  ExternalSaturationOutDataTypeStr=Inherit: Same as second input  DerivativeSourceVariant=Disabled  PreIntVariant=InternalPreInt
  Sum : Sum  Inputs=|+-
  Iqref : Outport  VectorParamsAs1DForOutWhenUnconnected=off
  wires:
  PIDController/1 -> Gain/1
  Gain/1 -> Iqref/1
  wmref/1 -> Sum/1
  Sum/1 -> PIDController/1
  wm/1 -> Sum/2

== system fix_FOC_sync/Subsystem3/Controller/FOC/abc2dq ==
  Iabc : Inport
  thetae : Inport  Port=2
  Demux1 : Demux  Outputs=3
  Park Transform : eeTransforms/Park Transform  AxisAlignment=D-axis  PowerInvariant=off
  Terminator : Terminator
  Id : Outport  VectorParamsAs1DForOutWhenUnconnected=off
  Iq : Outport  Port=2  VectorParamsAs1DForOutWhenUnconnected=off
  wires:
  Iabc/1 -> Park Transform/1
  thetae/1 -> Park Transform/2
  Demux1/3 -> Terminator/1
  Park Transform/1 -> Demux1/1
  Demux1/1 -> Id/1
  Demux1/2 -> Iq/1

== system fix_FOC_sync/Subsystem3/Controller/FOC/dq2abc ==
  Vd : Inport
  Vq : Inport  Port=2
  thetae : Inport  Port=3
  Constant : Constant  Value=0
  Inverse Park Transform : eeTransforms/Inverse Park Transform  AxisAlignment=D-axis  PowerInvariant=off
  Mux : Mux  Inputs=3
  Vabc : Outport  VectorParamsAs1DForOutWhenUnconnected=off
  wires:
  thetae/1 -> Inverse Park Transform/2
  Constant/1 -> Mux/3
  Mux/1 -> Inverse Park Transform/1
  Vd/1 -> Mux/1
  Inverse Park Transform/1 -> Vabc/1
  Vq/1 -> Mux/2

== system fix_FOC_sync/Subsystem3/Controller/FOC/thm2the ==
  thm : Inport
  Constant : Constant  Value=2*pi
  Mod : Math  Operator=mod  SignedPower=on
  PolePairs : Gain  Gain=p
  the : Outport  VectorParamsAs1DForOutWhenUnconnected=off
  wires:
  Constant/1 -> Mod/2
  PolePairs/1 -> Mod/1
  Mod/1 -> the/1
  thm/1 -> PolePairs/1

== system fix_FOC_sync/Subsystem3/Controller/FOC/wm2we ==
  wm : Inport
  PolePairs : Gain  Gain=p
  we : Outport  VectorParamsAs1DForOutWhenUnconnected=off
  wires:
  wm/1 -> PolePairs/1
  PolePairs/1 -> we/1

== system fix_FOC_sync/Subsystem4/Controller/DriverPeripherals/Break Algebraic Loop ==
  In1 : Inport
  Demux : Demux  Outputs=3
  Mux : Mux  Inputs=3
  Transfer Fcn : TransferFcn  Denominator=[1e-6 1]
  Transfer Fcn1 : TransferFcn  Denominator=[1e-6 1]
  Transfer Fcn2 : TransferFcn  Denominator=[1e-6 1]
  Out1 : Outport
  wires:
  In1/1 -> Demux/1
  Demux/1 -> Transfer Fcn/1
  Transfer Fcn/1 -> Mux/1
  Demux/2 -> Transfer Fcn1/1
  Transfer Fcn1/1 -> Mux/2
  Demux/3 -> Transfer Fcn2/1
  Transfer Fcn2/1 -> Mux/3
  Mux/1 -> Out1/1

== system fix_FOC_sync/Subsystem4/Controller/FOC/CurrentController ==
  Idref : Inport
  Iqref : Inport  Port=2
  Id : Inport  Port=3
  Iq : Inport  Port=4
  we : Inport  Port=5
  Decoupling : Subsystem
  IdController : slpidlib/PID Controller  Controller=PI  Form=Parallel  TimeDomain=Continuous-time  UseExternalTs=off  SampleTime=-1  IntegratorMethod=Forward Euler  FilterMethod=Forward Euler  ControllerParametersSource=internal  P=Kp_id  I=Ki_id  UseKiTs=off  D=0  UseExternalDerivativeSource=off  N=100  UseFilter=on  TunerSelectOption=Transfer Function Based (PID Tuner App)  InitialConditionSource=internal  InitialConditionForIntegrator=0  InitialConditionForFilter=0  DifferentiatorICPrevScaledInput=0  ExternalReset=none  TrackingMode=off  Kt=1  LimitOutput=off  SatLimitsSource=internal  UpperSaturationLimit=inf  LowerSaturationLimit=-inf  LinearizeAsGain=on  AntiWindupMode=none  Kb=1  LimitIntegrator=off  UpperIntegratorSaturationLimit=inf  LowerIntegratorSaturationLimit=-inf  POutMin=[]  POutMax=[]  IOutMin=[]  IOutMax=[]  DOutMin=[]  DOutMax=[]  NOutMin=[]  NOutMax=[]  SumOutMin=[]  SumOutMax=[]  SaturationOutMin=[]  SaturationOutMax=[]  PParamMin=[]  PParamMax=[]  IParamMin=[]  IParamMax=[]  DParamMin=[]  DParamMax=[]  NParamMin=[]  NParamMax=[]  KbParamMin=[]  KbParamMax=[]  KtParamMin=[]  KtParamMax=[]  KbOutMin=[]  KbOutMax=[]  KtOutMin=[]  KtOutMax=[]  IntegratorOutMin=[]  IntegratorOutMax=[]  FilterOutMin=[]  FilterOutMax=[]  SumI1OutMin=[]  SumI1OutMax=[]  SumI2OutMin=[]  SumI2OutMax=[]  SumI3OutMin=[]  SumI3OutMax=[]  SumI4OutMin=[]  SumI4OutMax=[]  SumDOutMin=[]  SumDOutMax=[]  DifferentiatorOutMin=[]  DifferentiatorOutMax=[]  FilterDiffOutCoefMin=[]  FilterDiffOutCoefMax=[]  ReciprocalOutMin=[]  ReciprocalOutMax=[]  SumDenOutMin=[]  SumDenOutMax=[]  SumNumOutMin=[]  SumNumOutMax=[]  DivideOutMin=[]  DivideOutMax=[]  UdiffTsProdOutMin=[]  UdiffTsProdOutMax=[]  NTsProdOutMin=[]  NTsProdOutMax=[]  UintegralTsProdOutMin=[]  UintegralTsProdOutMax=[]  UngainTsProdOutMin=[]  UngainTsProdOutMax=[]  ClampingZeroOutDataTypeStr=Inherit: Inherit via back propagation  ClampingZeroOutMin=[]  ClampingZeroOutMax=[]  FilterDenConstantOutDataTypeStr=Inherit: Inherit via back propagation  FilterDenConstantOutMin=[]  FilterDenConstantOutMax=[]  PCopyOutDataTypeStr=Inherit: Inherit via back propagation  PCopyOutMin=[]  PCopyOutMax=[]  NCopyOutDataTypeStr=Inherit: Inherit via back propagation  NCopyOutMin=[]  NCopyOutMax=[]  IntegratorContinuousStateAttributes=''  IntegratorStateMustResolveToSignalObject=off  IntegratorRTWStateStorageClass=Auto  FilterContinuousStateAttributes=''  FilterStateMustResolveToSignalObject=off  FilterRTWStateStorageClass=Auto  ParallelPVariant=InternalParameters  IdealPVariant=Disabled  IVariant=InternalParameters  DVariant=Disabled  IntegratorVariant=Continuous  SatVariant=Disabled  AWVariant=Passthrough  PCopyVariant=Disabled  TRVariant=Disabled  FdbkBlocksVariant=Forward  IdealPFdbkVariant=Disabled  SatFdbkVariant=Disabled  DerivativeFilterVariant=Disabled  NVariant=Disabled  NCopyVariant=Disabled_SignalSpec  FilterICVariant=Disabled  IntegratorICVariant=InternalICs  ExternalResetVariant=Disabled  TRSumVariant=Passthrough  SumFdbkVariant=Disabled  SumVariant=Sum_PI  TsampFilterVariant=InternalTs  TsampNgainVariant=Passthrough  TsampIntegralVariant=Disabled_SignalSpec  ExternalSaturationOutDataTypeStr=Inherit: Same as second input  DerivativeSourceVariant=Disabled  PreIntVariant=InternalPreInt
  IqController : slpidlib/PID Controller  Controller=PI  Form=Parallel  TimeDomain=Continuous-time  UseExternalTs=off  SampleTime=-1  IntegratorMethod=Forward Euler  FilterMethod=Forward Euler  ControllerParametersSource=internal  P=Kp_iq  I=Ki_iq  UseKiTs=off  D=0  UseExternalDerivativeSource=off  N=100  UseFilter=on  TunerSelectOption=Transfer Function Based (PID Tuner App)  InitialConditionSource=internal  InitialConditionForIntegrator=0  InitialConditionForFilter=0  DifferentiatorICPrevScaledInput=0  ExternalReset=none  TrackingMode=off  Kt=1  LimitOutput=off  SatLimitsSource=internal  UpperSaturationLimit=inf  LowerSaturationLimit=-inf  LinearizeAsGain=on  AntiWindupMode=none  Kb=1  LimitIntegrator=off  UpperIntegratorSaturationLimit=inf  LowerIntegratorSaturationLimit=-inf  POutMin=[]  POutMax=[]  IOutMin=[]  IOutMax=[]  DOutMin=[]  DOutMax=[]  NOutMin=[]  NOutMax=[]  SumOutMin=[]  SumOutMax=[]  SaturationOutMin=[]  SaturationOutMax=[]  PParamMin=[]  PParamMax=[]  IParamMin=[]  IParamMax=[]  DParamMin=[]  DParamMax=[]  NParamMin=[]  NParamMax=[]  KbParamMin=[]  KbParamMax=[]  KtParamMin=[]  KtParamMax=[]  KbOutMin=[]  KbOutMax=[]  KtOutMin=[]  KtOutMax=[]  IntegratorOutMin=[]  IntegratorOutMax=[]  FilterOutMin=[]  FilterOutMax=[]  SumI1OutMin=[]  SumI1OutMax=[]  SumI2OutMin=[]  SumI2OutMax=[]  SumI3OutMin=[]  SumI3OutMax=[]  SumI4OutMin=[]  SumI4OutMax=[]  SumDOutMin=[]  SumDOutMax=[]  DifferentiatorOutMin=[]  DifferentiatorOutMax=[]  FilterDiffOutCoefMin=[]  FilterDiffOutCoefMax=[]  ReciprocalOutMin=[]  ReciprocalOutMax=[]  SumDenOutMin=[]  SumDenOutMax=[]  SumNumOutMin=[]  SumNumOutMax=[]  DivideOutMin=[]  DivideOutMax=[]  UdiffTsProdOutMin=[]  UdiffTsProdOutMax=[]  NTsProdOutMin=[]  NTsProdOutMax=[]  UintegralTsProdOutMin=[]  UintegralTsProdOutMax=[]  UngainTsProdOutMin=[]  UngainTsProdOutMax=[]  ClampingZeroOutDataTypeStr=Inherit: Inherit via back propagation  ClampingZeroOutMin=[]  ClampingZeroOutMax=[]  FilterDenConstantOutDataTypeStr=Inherit: Inherit via back propagation  FilterDenConstantOutMin=[]  FilterDenConstantOutMax=[]  PCopyOutDataTypeStr=Inherit: Inherit via back propagation  PCopyOutMin=[]  PCopyOutMax=[]  NCopyOutDataTypeStr=Inherit: Inherit via back propagation  NCopyOutMin=[]  NCopyOutMax=[]  IntegratorContinuousStateAttributes=''  IntegratorStateMustResolveToSignalObject=off  IntegratorRTWStateStorageClass=Auto  FilterContinuousStateAttributes=''  FilterStateMustResolveToSignalObject=off  FilterRTWStateStorageClass=Auto  ParallelPVariant=InternalParameters  IdealPVariant=Disabled  IVariant=InternalParameters  DVariant=Disabled  IntegratorVariant=Continuous  SatVariant=Disabled  AWVariant=Passthrough  PCopyVariant=Disabled  TRVariant=Disabled  FdbkBlocksVariant=Forward  IdealPFdbkVariant=Disabled  SatFdbkVariant=Disabled  DerivativeFilterVariant=Disabled  NVariant=Disabled  NCopyVariant=Disabled_SignalSpec  FilterICVariant=Disabled  IntegratorICVariant=InternalICs  ExternalResetVariant=Disabled  TRSumVariant=Passthrough  SumFdbkVariant=Disabled  SumVariant=Sum_PI  TsampFilterVariant=InternalTs  TsampNgainVariant=Passthrough  TsampIntegralVariant=Disabled_SignalSpec  ExternalSaturationOutDataTypeStr=Inherit: Same as second input  DerivativeSourceVariant=Disabled  PreIntVariant=InternalPreInt
  Sum1 : Sum  Inputs=|+-
  Sum2 : Sum  Inputs=++|
  Sum3 : Sum  Inputs=++|
  Sum4 : Sum  Inputs=|+-
  Vdref : Outport  VectorParamsAs1DForOutWhenUnconnected=off
  Vqref : Outport  Port=2  VectorParamsAs1DForOutWhenUnconnected=off
  wires:
  we/1 -> Decoupling/3(we)
  Idref/1 -> Sum4/1
  Sum2/1 -> Vdref/1
  Sum3/1 -> Vqref/1
  Iqref/1 -> Sum1/1
  Iq/1 -> Decoupling/2(Iq), Sum1/2
  Id/1 -> Decoupling/1(Id), Sum4/2
  Sum4/1 -> IdController/1
  Sum1/1 -> IqController/1
  Decoupling/2(VqFF) -> Sum3/1
  Decoupling/1(VdFF) -> Sum2/1
  IdController/1 -> Sum2/2
  IqController/1 -> Sum3/2
